simulink model "AC_AC_voltage_controller"  (R2024b)
settings: Solver=VariableStepAuto  StartTime=0.0  StopTime=0.08  RelTol=1e-3
libraries: spsVoltageMeasurementLib x2, spsThyristorLib x2, spsACVoltageSourceLib x1, spsSeriesRLCBranchLib x1, sps_lib x1
settings Model: Creator=HARSH  LastModifiedBy=HARSH

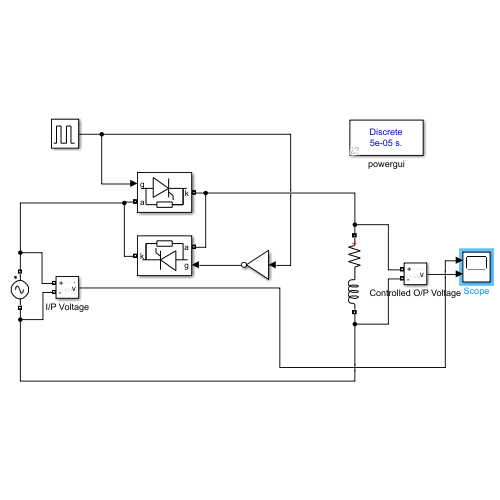
[thumbnail: Simulink's stored preview of the top-level diagram]
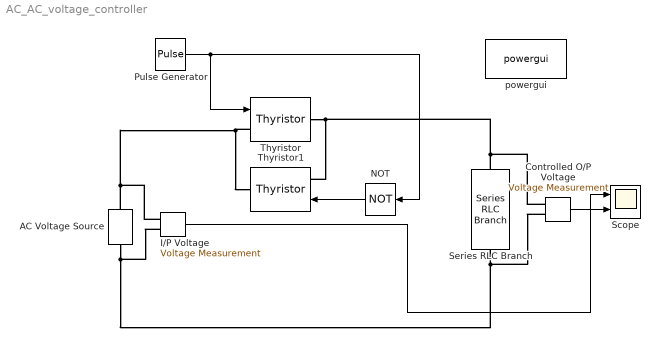
== system AC_AC_voltage_controller ==
  AC Voltage Source : spsACVoltageSourceLib/AC Voltage Source  Amplitude=100  Phase=0  Frequency=50  SampleTime=0  Measurements=None  BusType=swing  Pref=10e3  Qref=0  Qmin=-inf  Qmax=+inf
  Controlled O/P Voltage : spsVoltageMeasurementLib/Voltage Measurement  PhasorSimulation=off  OutputType=Complex  PSBequivalent=0
  I/P Voltage : spsVoltageMeasurementLib/Voltage Measurement  PhasorSimulation=off  OutputType=Complex  PSBequivalent=0
  NOT : Logic  Operator=NOT  IconShape=distinctive  AllPortsSameDT=off  OutDataTypeStr=boolean
  Pulse Generator : DiscretePulseGenerator  PulseType=Time based  Period=0.02  PulseWidth=50  PhaseDelay=1/500
  Scope : Scope  NumInputPorts=2
  Series RLC Branch : spsSeriesRLCBranchLib/Series RLC Branch  LConnTagsString=__new0  RConnTagsString=__new0  BranchType=RL  Resistance=50  Inductance=25e-3  SetiL0=off  InitialCurrent=0  Capacitance=1e-6  Setx0=off  InitialVoltage=0  Measurements=None
  Thyristor : spsThyristorLib/Thyristor  Ron=0.001  Lon=0  Vf=0.8  IC=0  Rs=500  Cs=250e-9  Measurements=off
  Thyristor1 : spsThyristorLib/Thyristor  Ron=0.001  Lon=0  Vf=0.8  IC=0  Rs=500  Cs=250e-9  Measurements=off
  powergui : sps_lib/powergui  Priority=1  SimulationMode=Discrete  SampleTime=50e-6  frequency=60  Iterations=50  frequencyindice=50  Pbase=100e6  ErrMax=1e-4  UnitsV=kV  UnitsW=MW  buscounter=0  FunctionMessages=off  echomessages=off  EnableUseOfTLC=off  CurrentSourceSwitches=off  DisableSnubberDevices=off  DisableRonSwitches=off  DisableVfSwitches=off  DisplayEquations=off  AutomaticDiscreteSolvers=off  SolverType=Tustin/Backward Euler (TBE)  Interpol=off  ExternalGateDelay=off  methode=off  Ts=100  x0status=blocks  SPID=on  SwTol=0  HookPort=off  NonlinearTolerance=1e-4  nMaxIteration=100  ContinueOnMaxIteration=off  RestoreLinks=warning  ResistiveCurrentMeasurement=off  Frange=[0:2:500]  Ylog=off  Xlog=on  ShowGrid=off  save=off  variable=ZData  structure=0  ZoomFFT=off  StartTime=0.0  cycles=1  DisplayStyle=1  fundamental=60  FreqAxis=off  MaxFrequency=1000  frequencyindicesteady=1  RmsSteady=1  display=off
  wires:
  Pulse Generator/1 -> NOT/1, Thyristor/1
  NOT/1 -> Thyristor1/1
  I/P Voltage/1 -> Scope/1
  Controlled O/P Voltage/1 -> Scope/2
  connections:
  Thyristor/LConn1 -- AC Voltage Source/RConn1 -- I/P Voltage/LConn1 -- Thyristor1/RConn1
  Thyristor/RConn1 -- Controlled O/P Voltage/LConn1 -- Series RLC Branch/LConn1 -- Thyristor1/LConn1
  AC Voltage Source/LConn1 -- I/P Voltage/LConn2 -- Controlled O/P Voltage/LConn2 -- Series RLC Branch/RConn1
